simulink model "AngleTracking"  (R2026b)
settings: Solver=VariableStepAuto
undefined symbols (not defined in the file): pllCfg
settings Model: Creator=24322  LastModifiedBy=24322

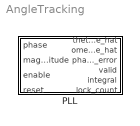
== system AngleTracking ==
  PLL : Subsystem  mask{pllCfg=pllCfg}
      mask prompts: pllCfg "PLL configuration"

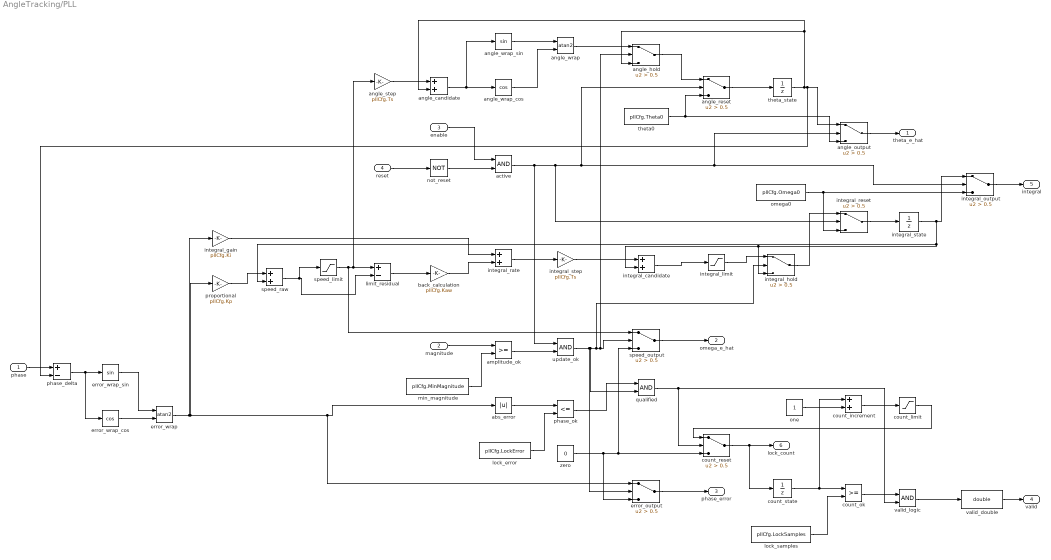
== system AngleTracking/PLL ==
  phase : Inport  SampleTime=pllCfg.Ts
  magnitude : Inport  Port=2  SampleTime=pllCfg.Ts
  enable : Inport  Port=3  SampleTime=pllCfg.Ts
  reset : Inport  Port=4  SampleTime=pllCfg.Ts
  abs_error : Abs  SaturateOnIntegerOverflow=off
  active : Logic  IconShape=distinctive  AllPortsSameDT=off  OutDataTypeStr=boolean
  amplitude_ok : RelationalOperator  OutDataTypeStr=boolean  RndMeth=Simplest  InputSameDT=off
  angle_candidate : Sum
  angle_hold : Switch  Criteria=u2 > Threshold  Threshold=0.5  SaturateOnIntegerOverflow=off  InputSameDT=off
  angle_output : Switch  Criteria=u2 > Threshold  Threshold=0.5  SaturateOnIntegerOverflow=off  InputSameDT=off
  angle_reset : Switch  Criteria=u2 > Threshold  Threshold=0.5  SaturateOnIntegerOverflow=off  InputSameDT=off
  angle_step : Gain  Gain=pllCfg.Ts
  angle_wrap : Trigonometry  Operator=atan2
  angle_wrap_cos : Trigonometry  Operator=cos
  angle_wrap_sin : Trigonometry
  back_calculation : Gain  Gain=pllCfg.Kaw
  count_increment : Sum
  count_limit : Saturate  UpperLimit=pllCfg.LockSamples  LowerLimit=0
  count_ok : RelationalOperator  OutDataTypeStr=boolean  RndMeth=Simplest  InputSameDT=off
  count_reset : Switch  Criteria=u2 > Threshold  Threshold=0.5  SaturateOnIntegerOverflow=off  InputSameDT=off
  count_state : UnitDelay  SampleTime=pllCfg.Ts
  error_output : Switch  Criteria=u2 > Threshold  Threshold=0.5  SaturateOnIntegerOverflow=off  InputSameDT=off
  error_wrap : Trigonometry  Operator=atan2
  error_wrap_cos : Trigonometry  Operator=cos
  error_wrap_sin : Trigonometry
  integral_candidate : Sum
  integral_gain : Gain  Gain=pllCfg.Ki
  integral_hold : Switch  Criteria=u2 > Threshold  Threshold=0.5  SaturateOnIntegerOverflow=off  InputSameDT=off
  integral_limit : Saturate  UpperLimit=pllCfg.OmegaMax  LowerLimit=-pllCfg.OmegaMax
  integral_output : Switch  Criteria=u2 > Threshold  Threshold=0.5  SaturateOnIntegerOverflow=off  InputSameDT=off
  integral_rate : Sum
  integral_reset : Switch  Criteria=u2 > Threshold  Threshold=0.5  SaturateOnIntegerOverflow=off  InputSameDT=off
  integral_state : UnitDelay  InitialCondition=pllCfg.Omega0  SampleTime=pllCfg.Ts
  integral_step : Gain  Gain=pllCfg.Ts
  limit_residual : Sum  Inputs=+-
  lock_error : Constant  Value=pllCfg.LockError
  lock_samples : Constant  Value=pllCfg.LockSamples
  min_magnitude : Constant  Value=pllCfg.MinMagnitude
  not_reset : Logic  Operator=NOT  IconShape=distinctive  AllPortsSameDT=off  OutDataTypeStr=boolean
  omega0 : Constant  Value=pllCfg.Omega0
  one : Constant
  phase_delta : Sum  Inputs=+-
  phase_ok : RelationalOperator  Operator=<=  OutDataTypeStr=boolean  RndMeth=Simplest  InputSameDT=off
  proportional : Gain  Gain=pllCfg.Kp
  qualified : Logic  IconShape=distinctive  AllPortsSameDT=off  OutDataTypeStr=boolean
  speed_limit : Saturate  UpperLimit=pllCfg.OmegaMax  LowerLimit=-pllCfg.OmegaMax
  speed_output : Switch  Criteria=u2 > Threshold  Threshold=0.5  SaturateOnIntegerOverflow=off  InputSameDT=off
  speed_raw : Sum
  theta0 : Constant  Value=pllCfg.Theta0
  theta_state : UnitDelay  InitialCondition=pllCfg.Theta0  SampleTime=pllCfg.Ts
  update_ok : Logic  IconShape=distinctive  AllPortsSameDT=off  OutDataTypeStr=boolean
  valid_double : DataTypeConversion  OutDataTypeStr=double  SaturateOnIntegerOverflow=off  RndMeth=Floor
  valid_logic : Logic  IconShape=distinctive  AllPortsSameDT=off  OutDataTypeStr=boolean
  zero : Constant  Value=0
  theta_e_hat : Outport
  omega_e_hat : Outport  Port=2
  phase_error : Outport  Port=3
  valid : Outport  Port=4
  integral : Outport  Port=5
  lock_count : Outport  Port=6
  wires:
  integral_output/1 -> integral/1
  valid_double/1 -> valid/1
  error_output/1 -> phase_error/1
  speed_output/1 -> omega_e_hat/1
  angle_output/1 -> theta_e_hat/1
  valid_logic/1 -> valid_double/1
  count_ok/1 -> valid_logic/1
  lock_samples/1 -> count_ok/2
  count_reset/1 -> count_state/1, lock_count/1
  qualified/1 -> count_reset/2, valid_logic/2
  count_limit/1 -> count_reset/1
  count_increment/1 -> count_limit/1
  one/1 -> count_increment/2
  count_state/1 -> count_increment/1, count_ok/1
  phase_ok/1 -> qualified/1
  lock_error/1 -> phase_ok/2
  abs_error/1 -> phase_ok/1
  zero/1 -> speed_output/3, count_reset/3, error_output/3
  integral_reset/1 -> integral_state/1
  angle_reset/1 -> theta_state/1
  omega0/1 -> integral_reset/3, integral_output/3
  integral_hold/1 -> integral_reset/1
  theta0/1 -> angle_reset/3, angle_output/3
  angle_hold/1 -> angle_reset/1
  integral_limit/1 -> integral_hold/1
  update_ok/1 -> angle_hold/2, speed_output/2, integral_hold/2, qualified/2, error_output/2
  angle_wrap/1 -> angle_hold/1
  angle_candidate/1 -> angle_wrap_sin/1, angle_wrap_cos/1
  angle_step/1 -> angle_candidate/1
  integral_candidate/1 -> integral_limit/1
  integral_step/1 -> integral_candidate/1
  integral_rate/1 -> integral_step/1
  back_calculation/1 -> integral_rate/2
  integral_gain/1 -> integral_rate/1
  limit_residual/1 -> back_calculation/1
  speed_limit/1 -> limit_residual/1, angle_step/1, speed_output/1
  speed_raw/1 -> speed_limit/1, limit_residual/2
  integral_state/1 -> integral_candidate/2, integral_hold/3, speed_raw/2, integral_output/1
  proportional/1 -> speed_raw/1
  error_wrap/1 -> error_output/1, abs_error/1, proportional/1, integral_gain/1
  phase_delta/1 -> error_wrap_sin/1, error_wrap_cos/1
  theta_state/1 -> phase_delta/2, angle_output/1, angle_candidate/2, angle_hold/3
  phase/1 -> phase_delta/1
  amplitude_ok/1 -> update_ok/2
  active/1 -> angle_output/2, integral_output/2, angle_reset/2, integral_reset/2, update_ok/1
  min_magnitude/1 -> amplitude_ok/2
  magnitude/1 -> amplitude_ok/1
  not_reset/1 -> active/2
  enable/1 -> active/1
  reset/1 -> not_reset/1
  angle_wrap_cos/1 -> angle_wrap/2
  angle_wrap_sin/1 -> angle_wrap/1
  error_wrap_cos/1 -> error_wrap/2
  error_wrap_sin/1 -> error_wrap/1
